simulink model "three_loop_deploy"  (R2023b)
settings: Solver=FixedStepDiscrete  StartTime=0  StopTime=1  FixedStep=5e-05  RelTol=1e-3
settings Model: Creator=92714  LastModifiedBy=92714
settings DataIOCC: SaveTime=off
settings OptimizationCC: DefaultParameterBehavior=Inlined  EnhancedBackFolding=on  PassReuseOutputArgsAs=Individual arguments  ZeroExternalMemoryAtStartup=off  ZeroInternalMemoryAtStartup=off  OptimizeBlockOrder=speed  DifferentSizesBufferReuse=on  OptimizationCustomize=off  EfficientTunableParamExpr=on
settings DebuggingCC: ParameterTunabilityLossMsg=error
settings HardwareCC: ProdBitPerPointer=32  ProdBitPerSizeT=32  ProdBitPerPtrDiffT=32  ProdLargestAtomicInteger=Long  ProdLargestAtomicFloat=Double  ProdWordSize=32  ProdHWDeviceType=ARM Compatible->ARM Cortex-M
settings SFSimCC: MATLABDynamicMemAlloc=off
settings RTWCC: Description=Embedded Coder  SystemTargetFile=ert.tlc  GenCodeOnly=on  GenerateMakefile=off  TemplateMakefile=ert_default_tmf  GenerateReport=on
settings CodeAppCC: ForceParamTrailComments=on  IgnoreCustomStorageClasses=off  OperatorAnnotations=on  SimulinkDataObjDesc=on  SFDataObjDesc=on  InsertBlockDesc=on
settings ERTTargetCC: TargetLangStandard=C99 (ISO)  IncludeMdlTerminateFcn=off  SuppressErrorStatus=on  SupportAbsoluteTime=off  SupportNonFinite=off  SupportComplex=off  InlinedParameterPlacement=NonHierarchical  ERTCustomFileTemplate=example_file_process.tlc

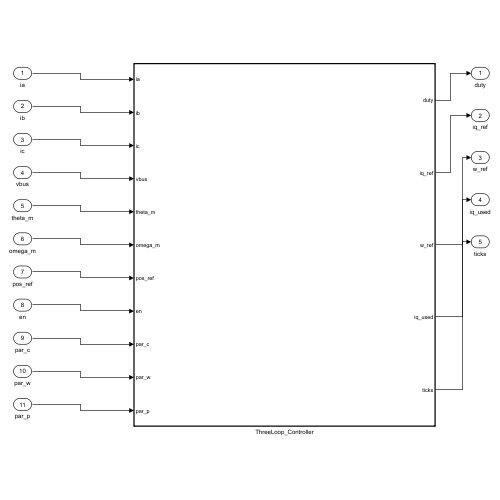
[thumbnail: Simulink's stored preview of the top-level diagram]
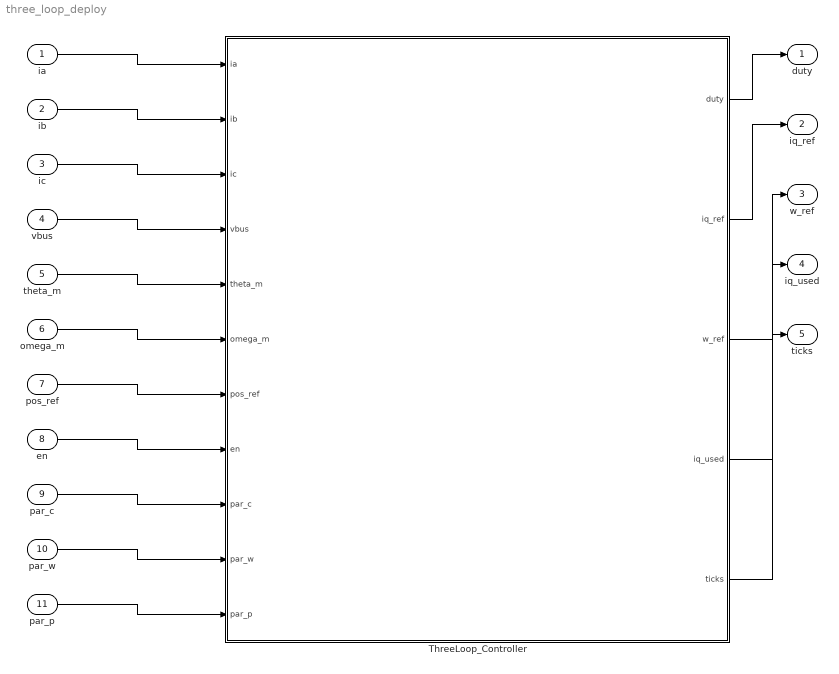
== system three_loop_deploy ==
  ia : Inport  OutDataTypeStr=single
  ib : Inport  Port=2  OutDataTypeStr=single
  ic : Inport  Port=3  OutDataTypeStr=single
  vbus : Inport  Port=4  OutDataTypeStr=single
  theta_m : Inport  Port=5  OutDataTypeStr=single
  omega_m : Inport  Port=6  OutDataTypeStr=single
  pos_ref : Inport  Port=7  OutDataTypeStr=single
  en : Inport  Port=8  OutDataTypeStr=single
  par_c : Inport  Port=9  OutDataTypeStr=single  PortDimensions=11
  par_w : Inport  Port=10  OutDataTypeStr=single  PortDimensions=5
  par_p : Inport  Port=11  OutDataTypeStr=single  PortDimensions=4
  ThreeLoop_Controller : Subsystem  TreatAsAtomicUnit=on
  duty : Outport
  iq_ref : Outport  Port=2
  w_ref : Outport  Port=3
  iq_used : Outport  Port=4
  ticks : Outport  Port=5
  wires:
  ia/1 -> ThreeLoop_Controller/1(ia)
  ib/1 -> ThreeLoop_Controller/2(ib)
  ic/1 -> ThreeLoop_Controller/3(ic)
  vbus/1 -> ThreeLoop_Controller/4(vbus)
  theta_m/1 -> ThreeLoop_Controller/5(theta_m)
  omega_m/1 -> ThreeLoop_Controller/6(omega_m)
  pos_ref/1 -> ThreeLoop_Controller/7(pos_ref)
  en/1 -> ThreeLoop_Controller/8(en)
  par_c/1 -> ThreeLoop_Controller/9(par_c)
  par_w/1 -> ThreeLoop_Controller/10(par_w)
  par_p/1 -> ThreeLoop_Controller/11(par_p)
  ThreeLoop_Controller/1(duty) -> duty/1
  ThreeLoop_Controller/2(iq_ref) -> iq_ref/1
  ThreeLoop_Controller/3(w_ref) -> w_ref/1
  ThreeLoop_Controller/4(iq_used) -> iq_used/1
  ThreeLoop_Controller/5(ticks) -> ticks/1

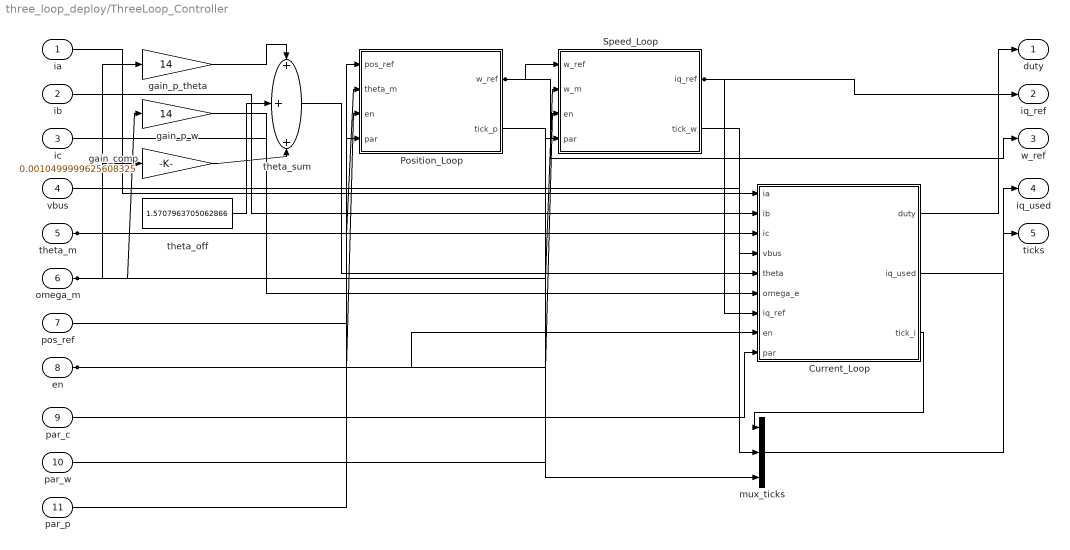
== system three_loop_deploy/ThreeLoop_Controller ==
  ia : Inport  OutDataTypeStr=single
  ib : Inport  Port=2  OutDataTypeStr=single
  ic : Inport  Port=3  OutDataTypeStr=single
  vbus : Inport  Port=4  OutDataTypeStr=single
  theta_m : Inport  Port=5  OutDataTypeStr=single
  omega_m : Inport  Port=6  OutDataTypeStr=single
  pos_ref : Inport  Port=7  OutDataTypeStr=single
  en : Inport  Port=8  OutDataTypeStr=single
  par_c : Inport  Port=9  OutDataTypeStr=single  PortDimensions=11
  par_w : Inport  Port=10  OutDataTypeStr=single  PortDimensions=5
  par_p : Inport  Port=11  OutDataTypeStr=single  PortDimensions=4
  Current_Loop : MATLAB Function  TreatAsAtomicUnit=on  SystemSampleTime=5e-05
  Position_Loop : MATLAB Function  TreatAsAtomicUnit=on  SystemSampleTime=5e-05
  Speed_Loop : MATLAB Function  TreatAsAtomicUnit=on  SystemSampleTime=5e-05
  gain_comp : Gain  Gain=0.0010499999625608325  ParamDataTypeStr=single  OutDataTypeStr=single
  gain_p_theta : Gain  Gain=14  ParamDataTypeStr=single  OutDataTypeStr=single
  gain_p_w : Gain  Gain=14  ParamDataTypeStr=single  OutDataTypeStr=single
  mux_ticks : Mux  Inputs=3
  theta_off : Constant  Value=1.5707963705062866  OutDataTypeStr=single
  theta_sum : Sum  Inputs=+++
  duty : Outport
  iq_ref : Outport  Port=2
  w_ref : Outport  Port=3
  iq_used : Outport  Port=4
  ticks : Outport  Port=5
  wires:
  theta_m/1 -> gain_p_theta/1, Position_Loop/2(theta_m)
  omega_m/1 -> gain_p_w/1, gain_comp/1, Speed_Loop/2(w_m)
  gain_p_theta/1 -> theta_sum/1
  theta_off/1 -> theta_sum/2
  gain_comp/1 -> theta_sum/3
  pos_ref/1 -> Position_Loop/1(pos_ref)
  en/1 -> Position_Loop/3(en), Speed_Loop/3(en), Current_Loop/8(en)
  par_p/1 -> Position_Loop/4(par)
  Position_Loop/1(w_ref) -> w_ref/1, Speed_Loop/1(w_ref)
  Position_Loop/2(tick_p) -> mux_ticks/3
  par_w/1 -> Speed_Loop/4(par)
  Speed_Loop/1(iq_ref) -> iq_ref/1, Current_Loop/7(iq_ref)
  Speed_Loop/2(tick_w) -> mux_ticks/2
  ia/1 -> Current_Loop/1(ia)
  ib/1 -> Current_Loop/2(ib)
  ic/1 -> Current_Loop/3(ic)
  vbus/1 -> Current_Loop/4(vbus)
  theta_sum/1 -> Current_Loop/5(theta)
  gain_p_w/1 -> Current_Loop/6(omega_e)
  par_c/1 -> Current_Loop/9(par)
  Current_Loop/1(duty) -> duty/1
  Current_Loop/2(iq_used) -> iq_used/1
  Current_Loop/3(tick_i) -> mux_ticks/1
  mux_ticks/1 -> ticks/1

== matlab function three_loop_deploy/ThreeLoop_Controller/Speed_Loop ==
  data: w_ref input; iq_ref output; w_m input; en input; par input; tick_w output
function [iq_ref, tick_w] = fcn_three_speed_loop_single(w_ref, w_m, en, par)
%FCN_THREE_SPEED_LOOP_SINGLE  速度环 PI（单精度 single 版，20 kHz ISR 内部分频 /10）
%
% 所有状态、常量、输出均为 single；积分步长 Ts_w=500us 不变。
% par = [kp_w, ki_w, Ts_w, i_max, N_div_w]

%#codegen
persistent i_term cnt hold_iq n_exec
if isempty(i_term)
    i_term   = single(0.0);
    cnt      = single(0.0);
    hold_iq  = single(0.0);
    n_exec   = single(0.0);
end

w_ref = single(w_ref);
w_m   = single(w_m);
en    = single(en);
par   = single(par);

kp    = par(1);
ki    = par(2);
ts    = par(3);
i_max = par(4);
n_div = par(5);

if en < single(0.5)
    i_term  = single(0.0);
    hold_iq = single(0.0);
else
    cnt = cnt + single(1.0);
    if cnt >= n_div
        cnt    = single(0.0);
        n_exec = n_exec + single(1.0);

        err = w_ref - w_m;
        i_term = i_term + ki * err * ts;
        if i_term > i_max
            i_term = i_max;
        elseif i_term < -i_max
            i_term = -i_max;
        end

        out = kp * err + i_term;
        if out > i_max
            out = i_max;
        elseif out < -i_max
            out = -i_max;
        end
        hold_iq = out;
    end
end

iq_ref = hold_iq;
tick_w = n_exec;
end

== matlab function three_loop_deploy/ThreeLoop_Controller/Position_Loop ==
  data: pos_ref input; w_ref output; theta_m input; en input; par input; tick_p output
function [w_ref, tick_p] = fcn_three_pos_loop_single(pos_ref, theta_m, en, par)
%FCN_THREE_POS_LOOP_SINGLE  位置环 P（单精度 single 版，20 kHz ISR 内部分频 /20）
%
% 所有状态、常量、输出均为 single；ERT 生成 real32_T + 无 double 软件库调用。
% 输入在开头显式转 single，兼容闭环 MIL 仿真中 double 的 plant/激励。
% par = [kp_p, w_max, Ts_p, N_div_p]

%#codegen
persistent cnt hold_w n_exec
if isempty(cnt)
    cnt    = single(0.0);
    hold_w = single(0.0);
    n_exec = single(0.0);
end

pos_ref = single(pos_ref);
theta_m = single(theta_m);
en      = single(en);
par     = single(par);

kp    = par(1);
w_max = par(2);
n_div = par(4);

if en < single(0.5)
    hold_w = single(0.0);
else
    cnt = cnt + single(1.0);
    if cnt >= n_div
        cnt    = single(0.0);
        n_exec = n_exec + single(1.0);
        w = kp * (pos_ref - theta_m);
        if w > w_max
            w = w_max;
        elseif w < -w_max
            w = -w_max;
        end
        hold_w = w;
    end
end

w_ref  = hold_w;
tick_p = n_exec;
end

== matlab function three_loop_deploy/ThreeLoop_Controller/Current_Loop ==
  data: ia input; duty output; ib input; ic input; vbus input; theta input; omega_e input; iq_ref input; en input; par input; iq_used output; tick_i output
function [duty, iq_used, tick_i] = fcn_three_current_loop_single(ia, ib, ic, vbus, theta, omega_e, iq_ref, en, par)
%FCN_THREE_CURRENT_LOOP_SINGLE  有感 FOC 电流环（单精度 single 版，20 kHz 每拍）
%
% 与 double 版逐行一致，仅把所有状态/常量/输出改为 single。
% ERT 生成 real32_T 变量 + sinf/cosf/sqrtf，M4F 硬件 FPU 可直接执行。
% par = [kp ki dt Ld Lq psi max_duty overmod mag_vd_max dec imax]

%#codegen
persistent vd_int vq_int n_exec
if isempty(vd_int)
    vd_int = single(0.0);
    vq_int = single(0.0);
    n_exec = single(0.0);
end
n_exec = n_exec + single(1.0);
tick_i = n_exec;

ia      = single(ia);
ib      = single(ib);
ic      = single(ic);
vbus    = single(vbus);
theta   = single(theta);
omega_e = single(omega_e);
iq_ref  = single(iq_ref);
en      = single(en);
par     = single(par);

kp         = par(1);
ki         = par(2);
dt         = par(3);
Ld         = par(4);
Lq         = par(5);
psi        = par(6);
max_duty   = par(7);
overmod    = par(8);
mag_vd_max = par(9);
dec_mode   = par(10);
i_max      = par(11);

ONE_BY_SQRT3 = single(0.5773502691896258);
TWO_BY_SQRT3 = single(1.1547005383792515);

% ---- Clarke（幅值不变）----
i_alpha = ia;
i_beta  = ONE_BY_SQRT3 * ia + TWO_BY_SQRT3 * ib;

s = sin(theta);
c = cos(theta);

% ---- Park（标准）----
id = c * i_alpha + s * i_beta;
iq = c * i_beta  - s * i_alpha;

% ---- 电流给定限幅 ----
iq_cmd = iq_ref;
if iq_cmd > i_max
    iq_cmd = i_max;
elseif iq_cmd < -i_max
    iq_cmd = -i_max;
end
iq_used = iq_cmd;

vd        = single(0.0);
vq        = single(0.0);
mod_alpha = single(0.0);
mod_beta  = single(0.0);
sector    = 0.0;
duty      = single([0.5; 0.5; 0.5]);

if en < single(0.5)
    vd_int = single(0.0);
    vq_int = single(0.0);
else
    err_d = single(0.0) - id;
    err_q = iq_cmd - iq;

    % 积分先行，再比例
    vd_int = vd_int + err_d * ki * dt;
    vq_int = vq_int + err_q * ki * dt;

    vd = vd_int + err_d * kp;
    vq = vq_int + err_q * kp;

    % ---- 解耦前馈（dec=3：交叉耦合 + BEMF）----
    dec_vd   = single(0.0);
    dec_vq   = single(0.0);
    dec_bemf = single(0.0);
    if dec_mode == single(1.0) || dec_mode == single(3.0)
        dec_vd = iq * omega_e * Lq;
        dec_vq = id * omega_e * Ld;
    end
    if dec_mode == single(2.0) || dec_mode == single(3.0)
        dec_bemf = omega_e * psi;
    end
    vd = vd - dec_vd;
    vq = vq + dec_vq + dec_bemf;

    % ---- 电压圆限幅（d 轴优先，积分器同步钳位）----
    max_v_mag = ONE_BY_SQRT3 * max_duty * vbus * overmod;
    lim_d = max_v_mag * mag_vd_max;

    if vd > lim_d
        vd = lim_d;
    elseif vd < -lim_d
        vd = -lim_d;
    end
    if vd_int > lim_d
        vd_int = lim_d;
    elseif vd_int < -lim_d
        vd_int = -lim_d;
    end

    tmp = max_v_mag * max_v_mag - vd * vd;
    if tmp > single(0.0)
        max_vq = sqrt(tmp);
    else
        max_vq = single(0.0);
    end
    if vq > max_vq
        vq = max_vq;
    elseif vq < -max_vq
        vq = -max_vq;
    end
    if vq_int > max_vq
        vq_int = max_vq;
    elseif vq_int < -max_vq
        vq_int = -max_vq;
    end

    % ---- 归一化：mod = v * 1.5 / vbus ----
    vn    = single(1.5) / vbus;
    mod_d = vd * vn;
    mod_q = vq * vn;

    % ---- 反 Park（标准）----
    mod_alpha = c * mod_d - s * mod_q;
    mod_beta  = c * mod_q + s * mod_d;

    [duty, sector] = three_svm_single(mod_alpha, mod_beta, max_duty);
end
end

% =======================================================================
function [duty, sector] = three_svm_single(alpha, beta, max_mod)
%THREE_SVM_SINGLE  SVPWM 六扇区（single 版）

ONE_BY_SQRT3 = single(0.5773502691896258);
TWO_BY_SQRT3 = single(1.1547005383792515);

if beta >= single(0.0)
    if alpha >= single(0.0)
        if ONE_BY_SQRT3 * beta > alpha
            sector = 2;
        else
            sector = 1;
        end
    else
        if -ONE_BY_SQRT3 * beta > alpha
            sector = 3;
        else
            sector = 2;
        end
    end
else
    if alpha >= single(0.0)
        if -ONE_BY_SQRT3 * beta > alpha
            sector = 5;
        else
            sector = 6;
        end
    else
        if ONE_BY_SQRT3 * beta > alpha
            sector = 4;
        else
            sector = 5;
        end
    end
end

dA = single(0.5);
dB = single(0.5);
dC = single(0.5);

if sector == 1
    t1 = alpha - ONE_BY_SQRT3 * beta;
    t2 = TWO_BY_SQRT3 * beta;
    dA = (single(1.0) + t1 + t2) * single(0.5);
    dB = dA - t1;
    dC = dB - t2;
elseif sector == 2
    t2 = alpha + ONE_BY_SQRT3 * beta;
    t3 = -alpha + ONE_BY_SQRT3 * beta;
    dB = (single(1.0) + t2 + t3) * single(0.5);
    dA = dB - t3;
    dC = dA - t2;
elseif sector == 3
    t3 = TWO_BY_SQRT3 * beta;
    t4 = -alpha - ONE_BY_SQRT3 * beta;
    dB = (single(1.0) + t3 + t4) * single(0.5);
    dC = dB - t3;
    dA = dC - t4;
elseif sector == 4
    t4 = -alpha + ONE_BY_SQRT3 * beta;
    t5 = -TWO_BY_SQRT3 * beta;
    dC = (single(1.0) + t4 + t5) * single(0.5);
    dB = dC - t5;
    dA = dB - t4;
elseif sector == 5
    t5 = -alpha - ONE_BY_SQRT3 * beta;
    t6 = alpha - ONE_BY_SQRT3 * beta;
    dC = (single(1.0) + t5 + t6) * single(0.5);
    dA = dC - t5;
    dB = dA - t6;
else
    t6 = -TWO_BY_SQRT3 * beta;
    t1 = alpha + ONE_BY_SQRT3 * beta;
    dA = (single(1.0) + t1 + t6) * single(0.5);
    dC = dA - t1;
    dB = dC - t6;
end

d_max = (single(1.0) + max_mod) * single(0.5);
if dA > d_max
    dA = d_max;
elseif dA < single(0.0)
    dA = single(0.0);
end
if dB > d_max
    dB = d_max;
elseif dB < single(0.0)
    dB = single(0.0);
end
if dC > d_max
    dC = d_max;
elseif dC < single(0.0)
    dC = single(0.0);
end

duty = [dA; dB; dC];
end
